simulink model "Bridge_Cycloconveter_R_Load"  (R2023b)
settings: Solver=VariableStepAuto  StartTime=0.0  StopTime=2.0  RelTol=1e-3
libraries: spsThyristorLib x8, spsACVoltageSourceLib x2, spsIdealSwitchLib x2, spsCurrentMeasurementLib x1, spsSeriesRLCBranchLib x1, spsVoltageMeasurementLib x1, sps_lib x1
settings Model: Creator=Anuj  LastModifiedBy=Anuj

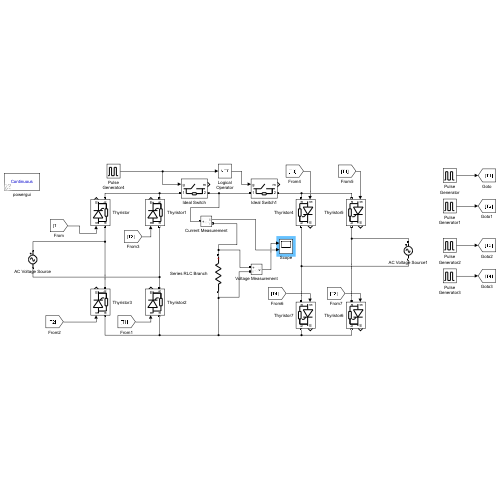
[thumbnail: Simulink's stored preview of the top-level diagram]
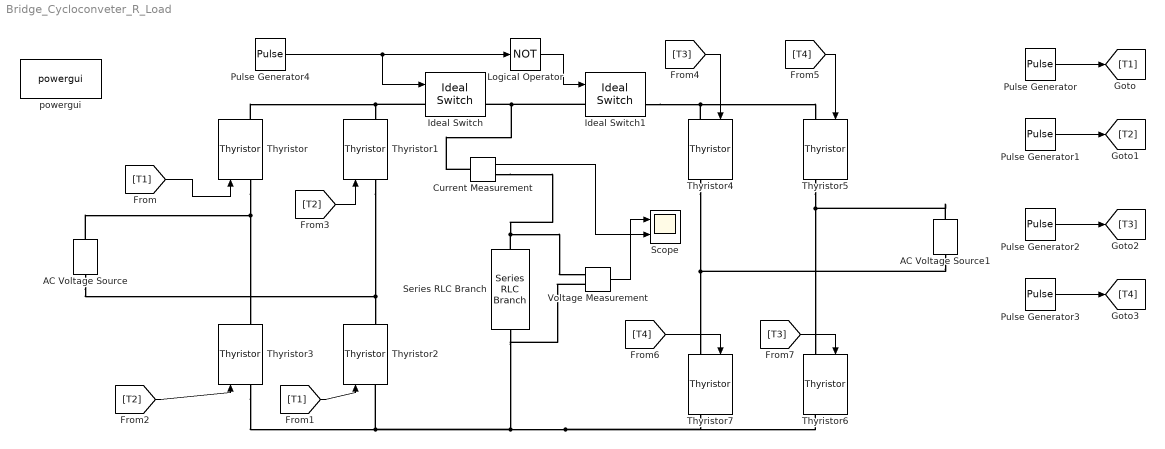
== system Bridge_Cycloconveter_R_Load ==
  AC Voltage Source : spsACVoltageSourceLib/AC Voltage Source  Amplitude=42.42  Phase=0  Frequency=50  SampleTime=0  Measurements=None  BusType=swing  Pref=10e3  Qref=0  Qmin=-inf  Qmax=+inf
  AC Voltage Source1 : spsACVoltageSourceLib/AC Voltage Source  Amplitude=42.42  Phase=0  Frequency=50  SampleTime=0  Measurements=None  BusType=swing  Pref=10e3  Qref=0  Qmin=-inf  Qmax=+inf
  Current Measurement : spsCurrentMeasurementLib/Current Measurement  PhasorSimulation=off  OutputType=Complex  PSBequivalent=0
  Ideal Switch : spsIdealSwitchLib/Ideal Switch  Ron=0.001  Lon=0  IC=0  Rs=1e5  Cs=inf  Measurements=on
  Ideal Switch1 : spsIdealSwitchLib/Ideal Switch  Ron=0.001  Lon=0  IC=0  Rs=1e5  Cs=inf  Measurements=on
  Logical Operator : Logic  Operator=NOT  AllPortsSameDT=off  OutDataTypeStr=boolean
  Pulse Generator : DiscretePulseGenerator  PulseType=Time based  Period=1/50  PulseWidth=50  PhaseDelay=0.02*(47/360)
  Pulse Generator1 : DiscretePulseGenerator  PulseType=Time based  Period=1/50  PulseWidth=50  PhaseDelay=0.02*((180+47)/360)
  Pulse Generator2 : DiscretePulseGenerator  PulseType=Time based  Period=1/50  PulseWidth=50  PhaseDelay=0.02*(47/360)
  Pulse Generator3 : DiscretePulseGenerator  PulseType=Time based  Period=1/50  PulseWidth=50  PhaseDelay=0.02*((180+47)/360)
  Pulse Generator4 : DiscretePulseGenerator  PulseType=Time based  Period=4/50  PulseWidth=50
  Scope : Scope  NumInputPorts=2
  Series RLC Branch : spsSeriesRLCBranchLib/Series RLC Branch  LConnTagsString=__new0  RConnTagsString=__new0  BranchType=R  Resistance=1  Inductance=1e-3  SetiL0=off  InitialCurrent=0  Capacitance=1e-6  Setx0=off  InitialVoltage=0  Measurements=None
  Thyristor{,1..7} (8 alike) : spsThyristorLib/Thyristor  Ron=0.001  Lon=0  Vf=0.8  IC=0  Rs=500  Cs=250e-9  Measurements=on
  Voltage Measurement : spsVoltageMeasurementLib/Voltage Measurement  PhasorSimulation=off  OutputType=Complex  PSBequivalent=0
  powergui : sps_lib/powergui  Priority=1  SimulationMode=Continuous  SampleTime=50e-6  frequency=60  Iterations=50  frequencyindice=50  Pbase=100e6  ErrMax=1e-4  UnitsV=kV  UnitsW=MW  buscounter=0  FunctionMessages=off  echomessages=off  EnableUseOfTLC=off  CurrentSourceSwitches=off  DisableSnubberDevices=off  DisableRonSwitches=off  DisableVfSwitches=off  DisplayEquations=off  AutomaticDiscreteSolvers=off  SolverType=Tustin/Backward Euler (TBE)  Interpol=off  ExternalGateDelay=off  methode=off  Ts=100  x0status=blocks  SPID=on  SwTol=0  HookPort=off  NonlinearTolerance=1e-4  nMaxIteration=100  ContinueOnMaxIteration=off  RestoreLinks=warning  ResistiveCurrentMeasurement=off  Frange=[0:2:500]  Ylog=off  Xlog=on  ShowGrid=off  save=off  variable=ZData  structure=0  ZoomFFT=off  StartTime=0.0  cycles=1  DisplayStyle=1  fundamental=60  FreqAxis=off  MaxFrequency=1000  frequencyindicesteady=1  RmsSteady=1  display=off
  wires:
  Current Measurement/1 -> Scope/2
  Voltage Measurement/1 -> Scope/1
  Pulse Generator/1 -> [T1]
  [T1] -> Thyristor/1
  [T1] -> Thyristor2/1
  Pulse Generator1/1 -> [T2]
  Pulse Generator2/1 -> [T3]
  Pulse Generator3/1 -> [T4]
  [T3] -> Thyristor4/1
  [T3] -> Thyristor6/1
  [T4] -> Thyristor5/1
  [T4] -> Thyristor7/1
  [T2] -> Thyristor3/1
  [T2] -> Thyristor1/1
  Pulse Generator4/1 -> Ideal Switch/1, Logical Operator/1
  Logical Operator/1 -> Ideal Switch1/1
  connections:
  Thyristor/LConn1 -- AC Voltage Source/RConn1 -- Thyristor3/RConn1
  Thyristor1/LConn1 -- AC Voltage Source/LConn1 -- Thyristor2/RConn1
  Thyristor/RConn1 -- Ideal Switch/LConn1 -- Thyristor1/RConn1
  Thyristor4/LConn1 -- Thyristor5/LConn1 -- Ideal Switch1/RConn1
  Thyristor4/RConn1 -- AC Voltage Source1/LConn1 -- Thyristor7/LConn1
  Thyristor5/RConn1 -- Thyristor6/LConn1 -- AC Voltage Source1/RConn1
  Thyristor3/LConn1 -- Voltage Measurement/LConn2 -- Series RLC Branch/RConn1 -- Thyristor7/RConn1 -- Thyristor6/RConn1 -- Thyristor2/LConn1
  Ideal Switch1/LConn1 -- Current Measurement/LConn1 -- Ideal Switch/RConn1
  Series RLC Branch/LConn1 -- Voltage Measurement/LConn1 -- Current Measurement/RConn1
